simulink model "LabB_TuneTheGyro"  (R2025b)
settings: Solver=FixedStepDiscrete  StartTime=0.0  StopTime=Inf  FixedStep=fSamplingPeriod  RelTol=1e-3  EnableMultiTasking=on
libraries: simulink x1
settings Model: SimulationMode=external  ExtModeTrigDuration=2  Creator=Alec  LastModifiedBy=abdgho
settings SolverCC: AlgebraicLoopSolver=TrustRegion
settings DataIOCC: LimitDataPoints=on  SaveFormat=Array  ReturnWorkspaceOutputs=off
settings OptimizationCC: PassReuseOutputArgsAs=Individual arguments  ExpressionDepthLimit=2147483647.0  MaxStackSize=64  EfficientTunableParamExpr=on
settings DebuggingCC: UnderspecifiedInitializationDetection=Classic  MergeDetectMultiDrivingBlocksExec=none  ParameterTunabilityLossMsg=error  UnconnectedInputMsg=warning  UnconnectedOutputMsg=warning  UnconnectedLineMsg=warning  StateNameClashWarn=warning  SFUnexpectedBacktrackingDiag=warning  SFNoUnconditionalDefaultTransitionDiag=warning  SFExecutionAtInitializationDiag=none  ArithmeticOperatorsInVariantConditions=warning
settings HardwareCC: ProdBitPerInt=16.0  ProdBitPerPointer=16.0  ProdBitPerSizeT=16.0  ProdBitPerPtrDiffT=16.0  ProdLargestAtomicFloat=None  ProdWordSize=8.0  ProdHWDeviceType=Atmel->AVR
settings ModelReferenceCC: EnableRefExpFcnMdlSchedulingChecks=on  PropagateSignalLabelsOutOfModel=off
settings SFSimCC: SimUseLocalCustomCode=off  MATLABDynamicMemAlloc=off  CustomCodeUndefinedFunction=UseInterfaceOnly
settings RTWCC: SystemTargetFile=ert.tlc  HardwareBoard=Arduino Mega 2560  TemplateMakefile=ert_default_tmf  GenerateReport=on  RTWVerbose=off  RTWUseLocalCustomCode=off  Toolchain=Arduino AVR  BuildConfiguration=Faster Runs  IncludeHyperlinkInReport=on  LaunchReport=on  GenerateTraceInfo=on  GenerateTraceReport=on  GenerateTraceReportSl=on  GenerateTraceReportSf=on  GenerateTraceReportEml=on  GPUComputeCapability=3.5  Description=Embedded Coder
settings CodeAppCC: ForceParamTrailComments=on  IgnoreCustomStorageClasses=off  OperatorAnnotations=on  SimulinkDataObjDesc=on  SFDataObjDesc=on  MATLABFcnDesc=on  CustomSymbolStrType=$N$R$M  InsertBlockDesc=on  StateflowObjectComments=on  MATLABSourceComments=on  InternalIdentifier=Classic
settings ERTTargetCC: InlinedParameterPlacement=Hierarchical  DynamicArrayContainerType=coder::array  SupportContinuousTime=on  SupportVariableSizeSignals=on
settings ConfigComp: CovMetricSettings=dw  CovSaveCumulativeToWorkspaceVar=on  CovSaveSingleToWorkspaceVar=on  CovExternalEMLEnable=off

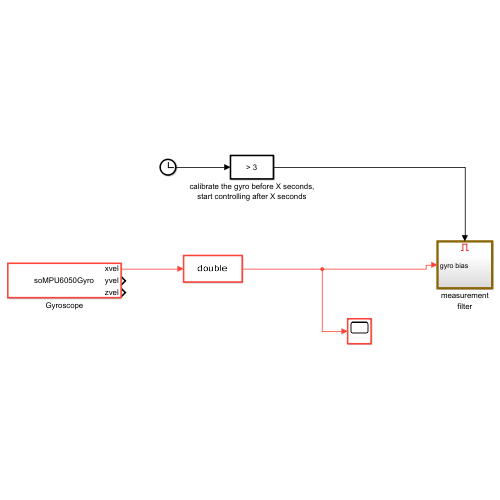
[thumbnail: Simulink's stored preview of the top-level diagram]
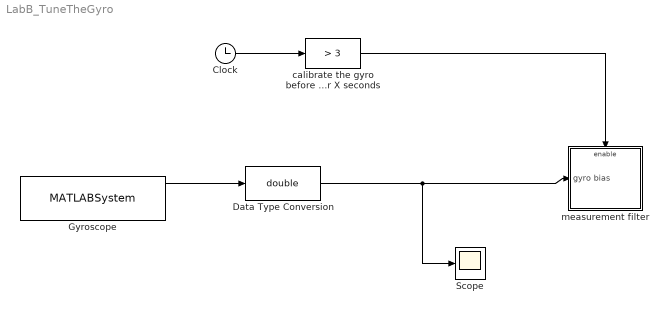
== system LabB_TuneTheGyro ==
  Clock : Clock
  Data Type Conversion : DataTypeConversion  OutDataTypeStr=double  SaturateOnIntegerOverflow=off  RndMeth=Floor
  Gyroscope : MATLABSystem  System=soMPU6050Gyro  DLPFmode=0
      mask Type: soMPU6050Gyro
  Scope : Scope
      settings: ActiveDisplayYMinimum=-1137.53125  ActiveDisplayYMaximum=653.84375  DataLoggingVariableName=gyroRawCalibration
  "calibrate the gyro before X seconds, start controlling after X seconds" : simulink/Logic and Bit Operations/Compare To Constant  relop=>  const=3  OutDataTypeStr=boolean
  measurement filter : Subsystem
  wires:
  Data Type Conversion/1 -> measurement filter/1(gyro bias), Scope/1
  Gyroscope/1 -> Data Type Conversion/1
  "calibrate the gyro before X seconds, start controlling after X seconds"/1 -> measurement filter/Enable
  Clock/1 -> "calibrate the gyro before X seconds, start controlling after X seconds"/1

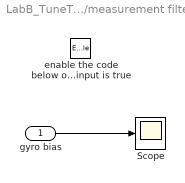
== system LabB_TuneTheGyro/measurement filter ==
  gyro bias : Inport
  "enable the code below only when the external boolean input is true " : EnablePort
  Scope : Scope
      settings: ActiveDisplayYMinimum=-17707.75  ActiveDisplayYMaximum=18119.75  DataLoggingVariableName=afGyroBias
  wires:
  gyro bias/1 -> Scope/1
